simulink model "DPS_LCupdated_discharging"  (R2025a)
settings: Solver=FixedStepAuto  StartTime=0.0  StopTime=0.3  FixedStep=1e-7  RelTol=1e-3
undefined symbols (not defined in the file): Ion, Lithium
libraries: spsSeriesRLCBranchLib x9, spsVoltageMeasurementLib x5, spsCurrentMeasurementLib x4, spsIGBTDiodeLib x4, spsMosfetLib x4, spsMeanLib x2, spsBatteryLib x1, spsDCVoltageSourceLib x1, spsLinearTransformerLib x1, sps_lib x1
settings Model: Creator=photortist  LastModifiedBy=photortist

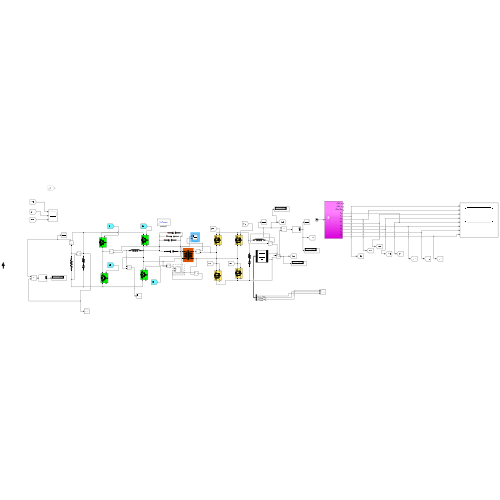
[thumbnail: Simulink's stored preview of the top-level diagram]
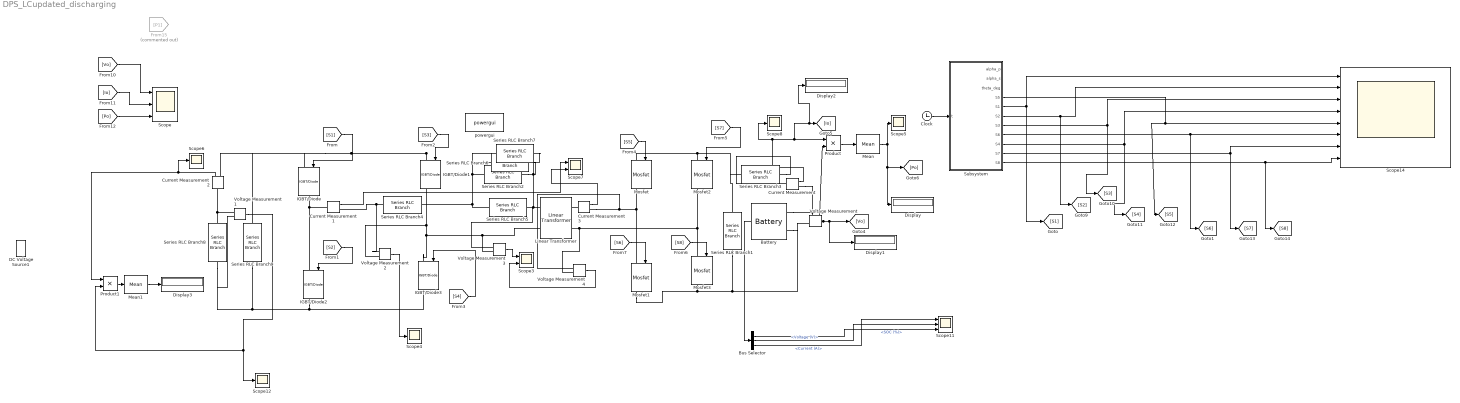
== system DPS_LCupdated_discharging ==
  Battery : spsBatteryLib/Battery  BatType=Lithium-Ion  NomV=24  NomQ=200  SOC=100  Batt_Tr=0.1  PresetModel=off  MaxQ=100  MinV=18  FullV=27.9357  Dis_rate=43.4783  R=0.0024  Normal_OP=90.4348  expZone="[25.9293      4.91304]"
  Bus Selector : BusSelector  OutputSignals=SOC (%),Voltage (V),Current (A)
  Clock : Clock
  Current Measurement{,1..3} (4 alike) : spsCurrentMeasurementLib/Current Measurement  PhasorSimulation=off  OutputType=Complex  PSBequivalent=0
  DC Voltage Source1 : spsDCVoltageSourceLib/DC Voltage Source  Amplitude=504  Measurements=None
  Display{,1..3} (4 alike) : Display
  From15 : From  Commented=on  GotoTag=P1
  IGBT/Diode : spsIGBTDiodeLib/IGBT//Diode  Ron=1e-4  Rs=1e5  Cs=inf  Measurements=off
  IGBT/Diode1 : spsIGBTDiodeLib/IGBT//Diode  Ron=1e-4  Rs=1e5  Cs=inf  Measurements=on
  IGBT/Diode2 : spsIGBTDiodeLib/IGBT//Diode  Ron=1e-4  Rs=1e5  Cs=inf  Measurements=on
  IGBT/Diode3 : spsIGBTDiodeLib/IGBT//Diode  Ron=1e-4  Rs=1e5  Cs=inf  Measurements=on
  Linear Transformer : spsLinearTransformerLib/Linear Transformer  UNITS=SI  NominalPower=[ 3000 30000 ]  winding1=[504 0 0]  winding2=[28 0 0]  ThreeWindings=off  winding3=[3.15e+05 0.7938 0.084225]  RmLm="[5000  0.05]"  Measurements=None  DataType=on
  Mean : spsMeanLib/Mean  Freq=30e3  Vinit=0  Ts=0
  Mean1 : spsMeanLib/Mean  Freq=30e3  Vinit=0  Ts=0
  Mosfet{,1..3} (4 alike) : spsMosfetLib/Mosfet  Ron=1e-4  Lon=0  Rd=0.01  Vfd=0  IC=0  Rs=1e5  Cs=inf  Measurements=on
  Product : Product
  Product1 : Product
  Scope : Scope  NumInputPorts=3
      settings: Title=Output Voltage  ActiveDisplayYMinimum=-3.1536  ActiveDisplayYMaximum=28.3823
  Scope11 : Scope  NumInputPorts=3
      settings: ActiveDisplayYMinimum=-185.34940276747079  ActiveDisplayYMaximum=453.55402462803829  DataLoggingVariableName=ScopeData11
  Scope{4..6,8,12} (5 alike) : Scope
      Scope12 settings: ActiveDisplayYMinimum=-68.267431635941051  ActiveDisplayYMaximum=614.4068847234696  DataLoggingVariableName=ScopeData12
      Scope4 settings: ActiveDisplayYMinimum=-630.0088  ActiveDisplayYMaximum=630.0088  DataLoggingVariableName=ScopeData4
      Scope5 settings: ActiveDisplayYMinimum=-393.1095  ActiveDisplayYMaximum=3537.9859  DataLoggingVariableName=ScopeData5
      Scope6 settings: ActiveDisplayYMinimum=-23.6358  ActiveDisplayYMaximum=24.8626  DataLoggingVariableName=ScopeData6
      Scope8 settings: ActiveDisplayYMinimum=-843.8589  ActiveDisplayYMaximum=389.6438  DataLoggingVariableName=ScopeData8
  Scope14 : Scope  NumInputPorts=8
      settings: ActiveDisplayYMinimum=-0.125  ActiveDisplayYMaximum=1.125  DataLoggingVariableName=ScopeData14
  Scope3 : Scope  NumInputPorts=2
      settings: ActiveDisplayYMinimum=-1589.4498571296351  ActiveDisplayYMaximum=1662.0755039892749  DataLoggingVariableName=ScopeData3
  Scope7 : Scope  NumInputPorts=2
      settings: Title=Overallcurrent  ActiveDisplayYMinimum=-248.66536425725388  ActiveDisplayYMaximum=249.02442247975975  YLabel=Input Current  DataLoggingVariableName=ScopeData7
  Series RLC Branch1 : spsSeriesRLCBranchLib/Series RLC Branch  LConnTagsString=__new0  RConnTagsString=__new0  BranchType=RC  Resistance=0.0002  Inductance=1e-3  SetiL0=off  InitialCurrent=0  Capacitance=1000e-6  Setx0=off  InitialVoltage=0  Measurements=None
  Series RLC Branch{2,5..7} (4 alike) : spsSeriesRLCBranchLib/Series RLC Branch  LConnTagsString=__new0  RConnTagsString=__new0  BranchType=C  Resistance=0.01  Inductance=350e-6  SetiL0=off  InitialCurrent=0  Capacitance=0.12e-6  Setx0=off  InitialVoltage=0  Measurements=None
  Series RLC Branch3 : spsSeriesRLCBranchLib/Series RLC Branch  LConnTagsString=__new0  RConnTagsString=__new0  BranchType=L  Resistance=7  Inductance=7e-6  SetiL0=off  InitialCurrent=0  Capacitance=1e-6  Setx0=off  InitialVoltage=0  Measurements=None
  Series RLC Branch4 : spsSeriesRLCBranchLib/Series RLC Branch  LConnTagsString=__new0  RConnTagsString=__new0  BranchType=L  Resistance=1  Inductance=80e-6  SetiL0=off  InitialCurrent=0  Capacitance=1e-6  Setx0=off  InitialVoltage=0  Measurements=None
  Series RLC Branch8 : spsSeriesRLCBranchLib/Series RLC Branch  LConnTagsString=__new0  RConnTagsString=__new0  BranchType=R  Resistance=85  Inductance=80e-6  SetiL0=off  InitialCurrent=0  Capacitance=1e-6  Setx0=off  InitialVoltage=0  Measurements=None
  Series RLC Branch9 : spsSeriesRLCBranchLib/Series RLC Branch  LConnTagsString=__new0  RConnTagsString=__new0  BranchType=RC  Resistance=0.002  Inductance=1e-3  SetiL0=off  InitialCurrent=0  Capacitance=1000e-6  Setx0=off  InitialVoltage=0  Measurements=None
  Subsystem : Subsystem
  Voltage Measurement{,1..4} (5 alike) : spsVoltageMeasurementLib/Voltage Measurement  PhasorSimulation=off  OutputType=Complex  PSBequivalent=0
  powergui : sps_lib/powergui  Priority=1  SimulationMode=Continuous  SampleTime=0.1e-6  frequency=60  Iterations=50  frequencyindice=0  Pbase=100e6  ErrMax=1e-4  UnitsV=kV  UnitsW=MW  buscounter=0  FunctionMessages=off  echomessages=off  EnableUseOfTLC=off  CurrentSourceSwitches=off  DisableSnubberDevices=off  DisableRonSwitches=off  DisableVfSwitches=off  DisplayEquations=off  AutomaticDiscreteSolvers=off  SolverType=Tustin/Backward Euler (TBE)  Interpol=off  ExternalGateDelay=off  methode=off  Ts=100  x0status=blocks  SPID=on  SwTol=0  HookPort=off  NonlinearTolerance=1e-4  nMaxIteration=100  ContinueOnMaxIteration=off  RestoreLinks=warning  ResistiveCurrentMeasurement=off  Frange=[0:2:500]  Ylog=off  Xlog=on  ShowGrid=off  save=off  variable=ZData  structure=0  ZoomFFT=off  StartTime=0.0  cycles=1  DisplayStyle=1  fundamental=60  FreqAxis=off  MaxFrequency=1000  frequencyindicesteady=1  RmsSteady=1  display=off
  wires:
  Current Measurement2/1 -> Product1/1, Scope6/1
  Product/1 -> Mean/1
  [Vo] -> Scope/1
  [S2] -> IGBT/Diode2/1
  [S4] -> IGBT/Diode3/1
  [S6] -> Mosfet1/1
  Mean1/1 -> Display3/1
  [S3] -> IGBT/Diode1/1
  Current Measurement3/1 -> Scope7/2
  Voltage Measurement2/1 -> Scope4/1
  [S8] -> Mosfet3/1
  Current Measurement/1 -> Scope8/1, Product/1, Display2/1, [Io]
  [Io] -> Scope/2
  [S7] -> Mosfet2/1
  Voltage Measurement3/1 -> Scope3/1
  [S1] -> IGBT/Diode/1
  Product1/1 -> Mean1/1
  Current Measurement1/1 -> Scope7/1
  [S5] -> Mosfet/1
  Voltage Measurement/1 -> Product/2, [Vo], Display1/1
  [Po] -> Scope/3
  Voltage Measurement4/1 -> Scope3/2
  Battery/1 -> Bus Selector/1
  Bus Selector/1 -> Scope11/3  "<SOC (%)>"
  Bus Selector/2 -> Scope11/2  "<Voltage (V)>"
  Bus Selector/3 -> Scope11/1  "<Current (A)>"
  Voltage Measurement1/1 -> Scope12/1, Product1/2
  Subsystem/7(S3) -> [S3], Scope14/3
  Subsystem/5(S1) -> [S1], Scope14/1
  Subsystem/6(S2) -> Scope14/2, [S2]
  Subsystem/11(S8) -> Scope14/8, [S8]
  Subsystem/9(S4) -> [S4], Scope14/4
  Subsystem/8(S6) -> [S6], Scope14/6
  Subsystem/4(S5) -> [S5], Scope14/5
  Subsystem/10(S7) -> [S7], Scope14/7
  Clock/1 -> Subsystem/1(t)
  Mean/1 -> Display/1, [Po], Scope5/1
  connections:
  Series RLC Branch8/LConn1 -- Current Measurement2/LConn1 -- Voltage Measurement1/LConn1
  Current Measurement3/RConn1 -- Voltage Measurement4/LConn1 -- Mosfet1/LConn1 -- Mosfet/RConn1
  Voltage Measurement2/LConn1 -- Current Measurement1/RConn1 -- Series RLC Branch4/LConn1
  Current Measurement/RConn1 -- Battery/LConn1 -- Voltage Measurement/LConn1
  Linear Transformer/RConn2 -- Mosfet3/LConn1 -- Mosfet2/RConn1 -- Voltage Measurement4/LConn2
  Linear Transformer/LConn2 -- IGBT/Diode3/LConn1 -- Voltage Measurement2/LConn2 -- IGBT/Diode1/RConn1 -- Voltage Measurement3/LConn2
  Series RLC Branch5/LConn1 -- Series RLC Branch7/LConn1 -- Series RLC Branch6/LConn1 -- Series RLC Branch2/LConn1 -- Series RLC Branch4/RConn1
  IGBT/Diode1/LConn1 -- Series RLC Branch9/LConn1 -- Current Measurement2/RConn1 -- IGBT/Diode/LConn1
  IGBT/Diode2/LConn1 -- IGBT/Diode/RConn1 -- Current Measurement1/LConn1
  Linear Transformer/LConn1 -- Series RLC Branch7/RConn1 -- Series RLC Branch6/RConn1 -- Series RLC Branch2/RConn1 -- Voltage Measurement3/LConn1 -- Series RLC Branch5/RConn1
  Linear Transformer/RConn1 -- Current Measurement3/LConn1
  Mosfet2/LConn1 -- Series RLC Branch3/LConn1 -- Series RLC Branch1/LConn1 -- Mosfet/LConn1
  Mosfet1/RConn1 -- Voltage Measurement/LConn2 -- Battery/LConn2 -- Series RLC Branch1/RConn1 -- Mosfet3/RConn1
  Series RLC Branch3/RConn1 -- Current Measurement/LConn1
  IGBT/Diode2/RConn1 -- Voltage Measurement1/LConn2 -- Series RLC Branch8/RConn1 -- Series RLC Branch9/RConn1 -- IGBT/Diode3/RConn1

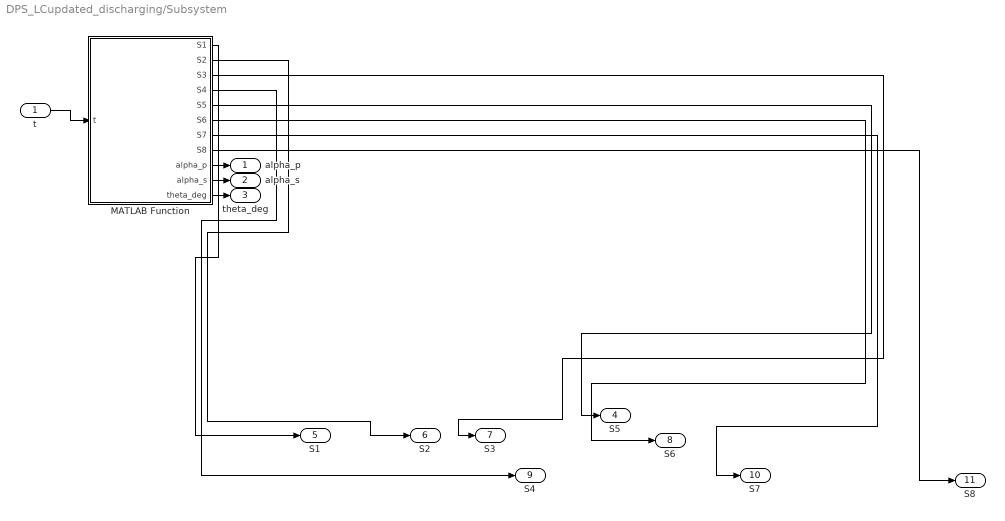
== system DPS_LCupdated_discharging/Subsystem ==
  t : Inport
  MATLAB Function : MATLAB Function  TreatAsAtomicUnit=on
  alpha_p : Outport
  alpha_s : Outport  Port=2
  theta_deg : Outport  Port=3
  S5 : Outport  Port=4
  S1 : Outport  Port=5
  S2 : Outport  Port=6
  S3 : Outport  Port=7
  S6 : Outport  Port=8
  S4 : Outport  Port=9
  S7 : Outport  Port=10
  S8 : Outport  Port=11
  wires:
  MATLAB Function/8(S8) -> S8/1
  MATLAB Function/2(S2) -> S2/1
  MATLAB Function/6(S6) -> S6/1
  MATLAB Function/7(S7) -> S7/1
  MATLAB Function/9(alpha_p) -> alpha_p/1
  MATLAB Function/3(S3) -> S3/1
  MATLAB Function/1(S1) -> S1/1
  MATLAB Function/5(S5) -> S5/1
  MATLAB Function/11(theta_deg) -> theta_deg/1
  MATLAB Function/4(S4) -> S4/1
  MATLAB Function/10(alpha_s) -> alpha_s/1
  t/1 -> MATLAB Function/1(t)

== matlab function DPS_LCupdated_discharging/Subsystem/MATLAB Function ==
  settings: updateMethod=DISCRETE
  data: S1 output; S2 output; S3 output; S4 output; S5 output; S6 output; S7 output; S8 output; t input; alpha_p output; alpha_s output; theta_deg output
function [S1, S2, S3, S4, S5, S6, S7, S8, alpha_p, alpha_s, theta_deg] = DAB_MaxPower_Test(t)
%#codegen
% =========================================================================
% FIXED MAXIMUM POWER TEST: alpha_p = 0 deg, alpha_s = 0 deg, theta = 90 deg
% Switching Frequency: fs = 30 kHz (Ts = 33.3333 us)
% =========================================================================

    % 1. FIXED ANGLES & DIRECTION
    alpha_p   =30 ;        % Primary inner shift = 0 deg
    alpha_s   =30;        % Secondary inner shift = 0 deg
    theta_deg =1;       % Outer phase shift = 90 deg (Max Power Point)
    DIRECTION = -1.0;        % +1.0 = HV -> LV, -1.0 = LV -> HV

    % 2. TIMING & DEAD-TIME PARAMETERS
    fs      = 30000.0;      % 30 kHz
    Ts      = 1.0 / fs;     % 33.3333 us
    half_Ts = Ts / 2.0;     % 180 deg = 16.6667 us

    dt_hv   = 0.2e-6;       % HV Dead-time = 0.4 us (Ideal test के लिए 0.0 कर सकते हैं)
    dt_lv   = 0.2e-6;       % LV Dead-time = 0.2 us

    % 3. CONVERT ANGLES TO TIME DELAYS
    theta_applied = DIRECTION * theta_deg;
    t_inner_hv    = ((2.0 * alpha_p) / 360.0) * Ts;   % 0 us
    t_inner_lv    = ((2.0 * alpha_s) / 360.0) * Ts;   % 0 us
    t_outer       = (theta_applied / 360.0) * Ts;     % 8.3333 us (Quarter period)

    % 4. CARRIER TIME REFERENCES
    t_hv_L = mod(t, Ts);                                    % HV Left Leg  (S1, S2)
    t_hv_R = mod(t - half_Ts - t_inner_hv, Ts);             % HV Right Leg (S3, S4)

    t_lv_L = mod(t - t_outer, Ts);                          % LV Left Leg  (S5, S6)
    t_lv_R = mod(t - t_outer - half_Ts - t_inner_lv, Ts);   % LV Right Leg (S7, S8)

    % 5. GATE PULSES (HV BRIDGE: S1..S4)
    if (t_hv_L >= dt_hv) && (t_hv_L < half_Ts), S1 = 1; else, S1 = 0; end
    if (t_hv_L >= half_Ts + dt_hv) && (t_hv_L < Ts), S2 = 1; else, S2 = 0; end

    if (t_hv_R >= dt_hv) && (t_hv_R < half_Ts), S3 = 1; else, S3 = 0; end
    if (t_hv_R >= half_Ts + dt_hv) && (t_hv_R < Ts), S4 = 1; else, S4 = 0; end

    % 6. GATE PULSES (LV BRIDGE: S5..S8)
    if (t_lv_L >= dt_lv) && (t_lv_L < half_Ts), S5 = 1; else, S5 = 0; end
    if (t_lv_L >= half_Ts + dt_lv) && (t_lv_L < Ts), S6 = 1; else, S6 = 0; end

    if (t_lv_R >= dt_lv) && (t_lv_R < half_Ts), S7 = 1; else, S7 = 0; end
    if (t_lv_R >= half_Ts + dt_lv) && (t_lv_R < Ts), S8 = 1; else, S8 = 0; end

end
